simulink model "Bilanciamento_MPC"  (R2026b)
settings: Solver=FixedStepDiscrete  StartTime=0  StopTime=par_sim.t_fine  FixedStep=par_sim.Tint
PostLoadFcn:
  | addpath(genpath(fileparts(fileparts(get_param('Bilanciamento_MPC', 'FileName')))));
  | if ~evalin('base', 'exist(''par_sim'', ''var'')')
  |     assignin('base', 'par_sim', parametri_simulazione());
  | end
InitFcn:
  | addpath(genpath(fileparts(fileparts(get_param('Bilanciamento_MPC', 'FileName')))));
  | if ~evalin('base', 'exist(''par_sim'', ''var'')')
  |     assignin('base', 'par_sim', parametri_simulazione());
  | end
values from neighbouring files (symbols this model uses):
  par_sim = parametri_simulazione(par, pacco, formulazione, par.(['scenario' scenario]), orizzonte)    [avvio_simulink.m]    (also in simula_simulink.m = parametri_simulazione(par, pacco, tipo, scen, p))
libraries: simulink x2
settings Model: Creator=Acer  LastModifiedBy=Acer

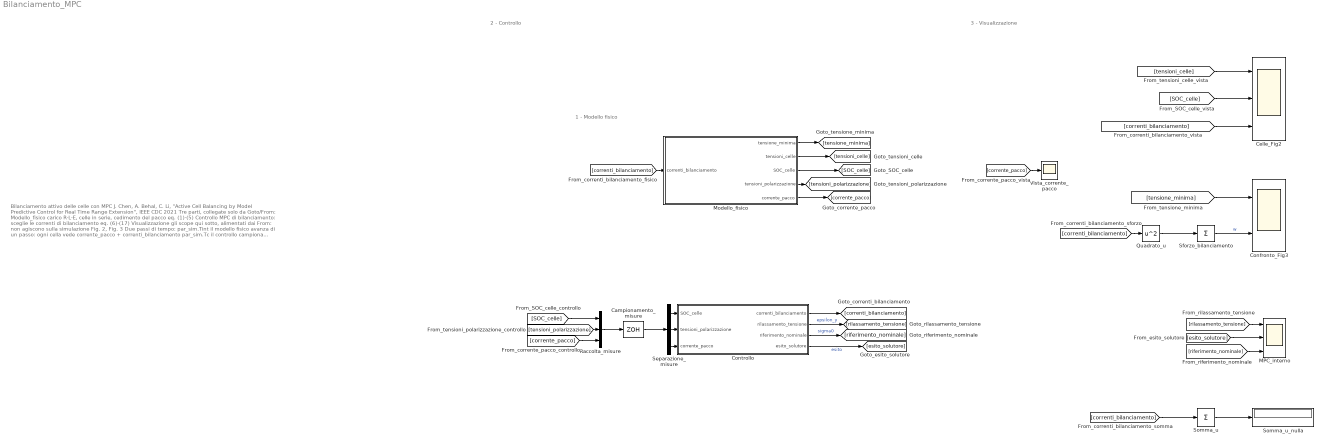
== system Bilanciamento_MPC ==
  note: Bilanciamento attivo delle celle con MPC
      | J. Chen, A. Behal, C. Li, "Active Cell Balancing by Model Predictive Control for Real Time Range Extension", IEEE CDC 2021
      |
      | Tre parti, collegate solo da Goto/From:
      |    Modello_fisico     carico R-L-E, celle in serie, cedimento del pacco             eq. (1)-(5)
      |    Controllo          MPC di bilanciamento: sceglie le correnti di bilanciamento    eq. (6)-(17)
      |    Visualizzazione    gli scope qui sotto, alimentati dai From: non agiscono sulla simulazione   Fig. 2, Fig. 3
      |
      | Due passi di tempo:
      |    par_sim.Tint         il modello fisico avanza di un passo: ogni cella vede corrente_pacco + correnti_bilanciamento
      |    par_sim.Tc           il controllo campiona corrente_pacco, SOC_celle e tensioni_polarizzazione e sceglie correnti_bilanciamento,
      |                         che restano costanti fino al passo di controllo successivo
      | La simulazione si ferma quando una cella scende sotto y_min.
      |
      | Parametri della simulazione nella struct 'par_sim' (avvio_simulink.m).
      | par_sim.n_J: 1 = J_t   2 = J_m   3 = J_Delta.  Confronto dei quattro casi: main_simulink.m
  note: 1 - Modello fisico
  note: 2 - Controllo
  note: 3 - Visualizzazione
  Campionamento_misure : ZeroOrderHold  SampleTime=par_sim.Tc
      settings: AttributesFormatString=ogni Tc
  Celle_Fig2 : Scope  NumInputPorts=3
      settings: AttributesFormatString=Fig. 2: y, s, u  ActiveDisplayString=3  Title=Corrente di bilanciamento u^n [A]  ActiveDisplayYMinimum=-2.4917702044223984  ActiveDisplayYMaximum=2.42593183980159
  Confronto_Fig3 : Scope  NumInputPorts=2
      settings: AttributesFormatString=Fig. 3: min y, sforzo w  Title=Sforzo di bilanciamento e_k = u_k'u_k [A^2]  ActiveDisplayYMinimum=0.52817346836693146  ActiveDisplayYMaximum=4.5629080222727767  DataLoggingVariableName=ScopeData2
  Controllo : Subsystem
      settings: AttributesFormatString=MPC: problema (6) risolto\ncome QP (Remark 3)
  MPC_interno : Scope  NumInputPorts=3
      settings: AttributesFormatString=epsilon_y, esito, sigma0  ActiveDisplayString=3  Title=Riferimento della cella nominale sigma0, eq. (7): una linea per passo dell'orizzonte  ActiveDisplayYMinimum=3.7199020855689335  ActiveDisplayYMaximum=4.2453442127145626
  Modello_fisico : Subsystem
      settings: AttributesFormatString=carico, celle, cedimento\neq. (1)-(5)
  Quadrato_u : Math  Operator=square
  Raccolta_misure : Mux  Inputs=[par_sim.N par_sim.N 1]
  Separazione_misure : Demux  Outputs=[par_sim.N par_sim.N 1]
  Sforzo_bilanciamento : Sum  Inputs=+
  Somma_u : Sum  Inputs=+
      settings: AttributesFormatString=eq. (6f)
  Somma_u_nulla : Display
      settings: AttributesFormatString=deve restare 0
  Vista_corrente_pacco : Scope
      settings: ActiveDisplayYMinimum=-2.0757062717769164  ActiveDisplayYMaximum=18.68135644599225  DataLoggingVariableName=ScopeData3
  wires:
  [correnti_bilanciamento] -> Quadrato_u/1
  Quadrato_u/1 -> Sforzo_bilanciamento/1
  [correnti_bilanciamento] -> Somma_u/1
  [correnti_bilanciamento] -> Celle_Fig2/3
  [riferimento_nominale] -> MPC_interno/3
  [esito_solutore] -> MPC_interno/2
  [SOC_celle] -> Celle_Fig2/2
  [rilassamento_tensione] -> MPC_interno/1
  [tensioni_celle] -> Celle_Fig2/1
  Sforzo_bilanciamento/1 -> Confronto_Fig3/2  "w"
  [tensione_minima] -> Confronto_Fig3/1
  Somma_u/1 -> Somma_u_nulla/1
  Controllo/4(esito_solutore) -> [esito_solutore]  "esito"
  Controllo/3(riferimento_nominale) -> [riferimento_nominale]  "sigma0"
  Controllo/2(rilassamento_tensione) -> [rilassamento_tensione]  "epsilon_y"
  Controllo/1(correnti_bilanciamento) -> [correnti_bilanciamento]
  Modello_fisico/5(corrente_pacco) -> [corrente_pacco]
  Modello_fisico/4(tensioni_polarizzazione) -> [tensioni_polarizzazione]
  Modello_fisico/3(SOC_celle) -> [SOC_celle]
  Modello_fisico/2(tensioni_celle) -> [tensioni_celle]
  Modello_fisico/1(tensione_minima) -> [tensione_minima]
  [correnti_bilanciamento] -> Modello_fisico/1(correnti_bilanciamento)
  [corrente_pacco] -> Vista_corrente_pacco/1
  [tensioni_polarizzazione] -> Raccolta_misure/2
  [SOC_celle] -> Raccolta_misure/1
  [corrente_pacco] -> Raccolta_misure/3
  Raccolta_misure/1 -> Campionamento_misure/1
  Campionamento_misure/1 -> Separazione_misure/1
  Separazione_misure/3 -> Controllo/3(corrente_pacco)
  Separazione_misure/2 -> Controllo/2(tensioni_polarizzazione)
  Separazione_misure/1 -> Controllo/1(SOC_celle)

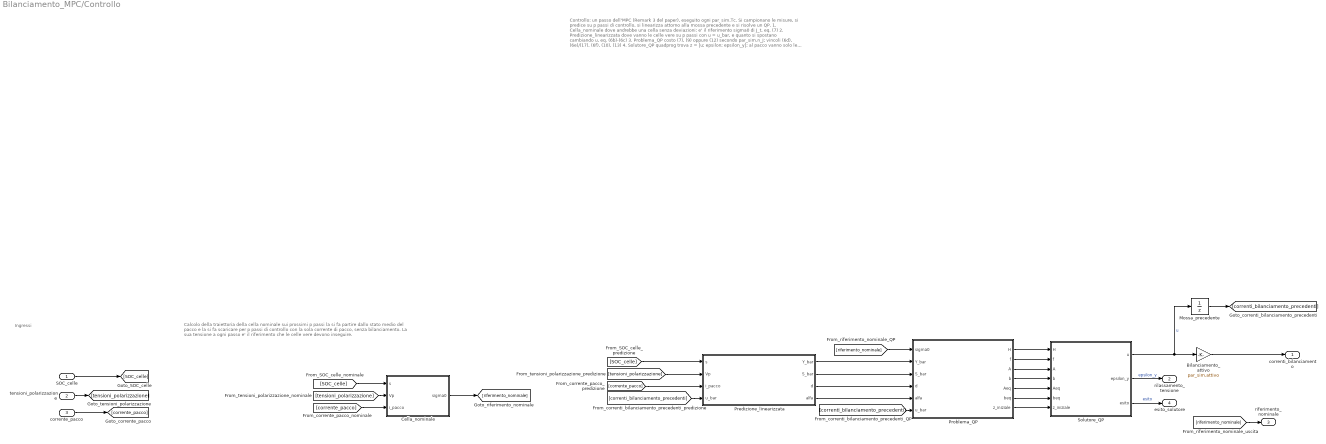
== system Bilanciamento_MPC/Controllo ==
  note: Ingressi
  note: Calcolo della traiettoria della cella nominale sui prossimi p passi
      |
      | la si fa partire dallo stato medio del pacco e la si fa scaricare per p passi di controllo con la sola corrente di pacco, senza bilanciamento.
      | La sua tensione a ogni passo e' il riferimento che le celle vere devono inseguire.
  note: Controllo: un passo dell'MPC (Remark 3 del paper), eseguito ogni par_sim.Tc. Si campionano le misure, si predice su p passi di controllo,
      | si linearizza attorno alla mossa precedente e si risolve un QP.
      |
      | 1. Cella_nominale            dove andrebbe una cella senza deviazioni: e' il riferimento sigma0 di J_t, eq. (7)
      | 2. Predizione_linearizzata   dove vanno le celle vere su p passi con u = u_bar, e quanto si spostano cambiando u, eq. (6b)-(6c)
      | 3. Problema_QP               costo (7), (9) oppure (12) secondo par_sim.n_J; vincoli (6d), (6e)/(17), (6f), (10), (13)
      | 4. Solutore_QP               quadprog trova z = [u; epsilon; epsilon_y]; al pacco vanno solo le u (orizzonte mobile)
      | 5. Bilanciamento_attivo      guadagno par_sim.attivo: con 0 il pacco lavora senza bilanciamento
      |
      | Doppio clic su un blocco per leggerne il codice; il calcolo vero e' nel file qp_*.m indicato nel commento.
  SOC_celle : Inport
  tensioni_polarizzazione : Inport  Port=2
  corrente_pacco : Inport  Port=3
  Bilanciamento_attivo : Gain  Gain=par_sim.attivo
      settings: AttributesFormatString=par_sim.attivo: 0 o 1
  Cella_nominale : MATLAB Function  TreatAsAtomicUnit=on
      settings: AttributesFormatString=eq. (7): riferimento sigma0
  Mossa_precedente : UnitDelay  InitialCondition=zeros(par_sim.N, 1)  SampleTime=par_sim.Tc
      settings: AttributesFormatString=u_bar = u_(k-1)
  Predizione_linearizzata : MATLAB Function  TreatAsAtomicUnit=on
      settings: AttributesFormatString=eq. (6b)-(6c), Remark 3
  Problema_QP : MATLAB Function  TreatAsAtomicUnit=on
      settings: AttributesFormatString=costo (7)/(9)/(12) e vincoli
  Solutore_QP : MATLAB Function  TreatAsAtomicUnit=on
      settings: AttributesFormatString=quadprog
  correnti_bilanciamento : Outport
  rilassamento_tensione : Outport  Port=2
  riferimento_nominale : Outport  Port=3
  esito_solutore : Outport  Port=4
  wires:
  corrente_pacco/1 -> [corrente_pacco]
  [corrente_pacco] -> Predizione_linearizzata/3(i_pacco)
  [tensioni_polarizzazione] -> Predizione_linearizzata/2(Vp)
  [SOC_celle] -> Predizione_linearizzata/1(s)
  [corrente_pacco] -> Cella_nominale/3(i_pacco)
  [tensioni_polarizzazione] -> Cella_nominale/2(Vp)
  [SOC_celle] -> Cella_nominale/1(s)
  Cella_nominale/1(sigma0) -> [riferimento_nominale]
  Predizione_linearizzata/1(Y_bar) -> Problema_QP/2(Y_bar)
  Predizione_linearizzata/2(S_bar) -> Problema_QP/3(S_bar)
  Predizione_linearizzata/3(d) -> Problema_QP/4(d)
  Predizione_linearizzata/4(alfa) -> Problema_QP/5(alfa)
  Problema_QP/1(H) -> Solutore_QP/1(H)
  Problema_QP/2(f) -> Solutore_QP/2(f)
  Problema_QP/3(A) -> Solutore_QP/3(A)
  Problema_QP/4(b) -> Solutore_QP/4(b)
  Problema_QP/5(Aeq) -> Solutore_QP/5(Aeq)
  Problema_QP/6(beq) -> Solutore_QP/6(beq)
  Problema_QP/7(z_iniziale) -> Solutore_QP/7(z_iniziale)
  [correnti_bilanciamento_precedenti] -> Predizione_linearizzata/4(u_bar)
  [correnti_bilanciamento_precedenti] -> Problema_QP/6(u_bar)
  Mossa_precedente/1 -> [correnti_bilanciamento_precedenti]
  Bilanciamento_attivo/1 -> correnti_bilanciamento/1
  Solutore_QP/1(u) -> Mossa_precedente/1, Bilanciamento_attivo/1  "u"
  tensioni_polarizzazione/1 -> [tensioni_polarizzazione]
  SOC_celle/1 -> [SOC_celle]
  [riferimento_nominale] -> riferimento_nominale/1
  [riferimento_nominale] -> Problema_QP/1(sigma0)
  Solutore_QP/2(epsilon_y) -> rilassamento_tensione/1  "epsilon_y"
  Solutore_QP/3(esito) -> esito_solutore/1  "esito"

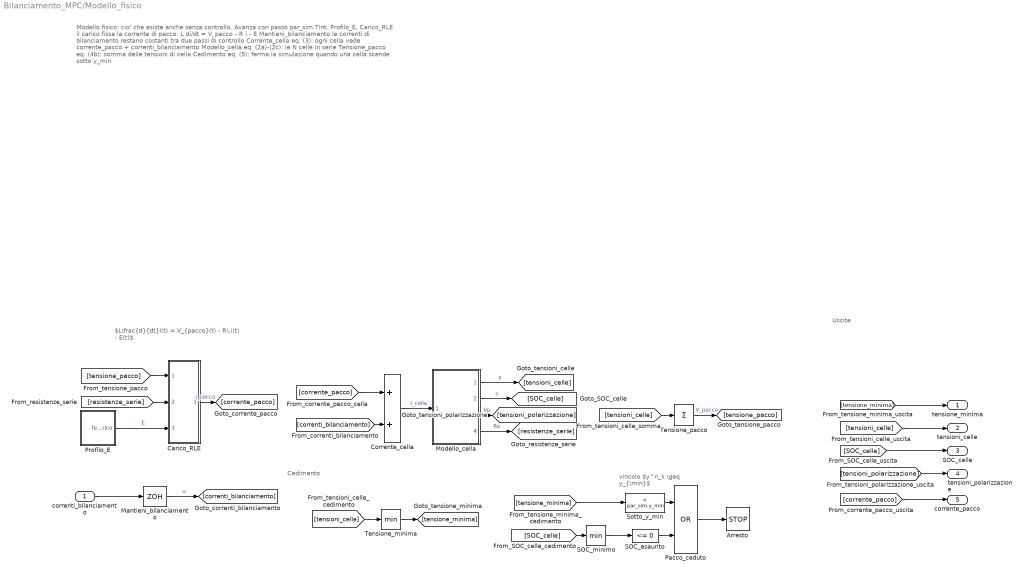
== system Bilanciamento_MPC/Modello_fisico ==
  note: vincolo $y^n_k \geq y_{\min}$
  note: $L\frac{d}{dt}i(t) = V_{pacco}(t) - R\,i(t) - E(t)$
  note: Cedimento
  note: Uscite
  note: Modello fisico: cio' che esiste anche senza controllo. Avanza con passo par_sim.Tint.
      |
      |    Profilo_E, Carico_RLE   il carico fissa la corrente di pacco:  L di/dt = V_pacco - R i - E
      |    Mantieni_bilanciamento  le correnti di bilanciamento restano costanti tra due passi di controllo
      |    Corrente_cella          eq. (3): ogni cella vede corrente_pacco + correnti_bilanciamento
      |    Modello_cella           eq. (2a)-(2c): le N celle in serie
      |    Tensione_pacco          eq. (4b): somma delle tensioni di cella
      |    Cedimento               eq. (5): ferma la simulazione quando una cella scende sotto y_min
  correnti_bilanciamento : Inport
  Arresto : Stop
  Carico_RLE : Subsystem
      settings: AttributesFormatString=L di_pacco/dt = V_pacco - R i_pacco - E
  Corrente_cella : Sum
      settings: AttributesFormatString=eq. (3): I_cella = i_pacco + u
  Mantieni_bilanciamento : ZeroOrderHold  SampleTime=par_sim.Tint
      settings: AttributesFormatString=costante tra due passi\ndi controllo
  Modello_cella : Subsystem
      settings: AttributesFormatString=eq. (2a)-(2c), (4a)
  Pacco_ceduto : Logic  Operator=OR  AllPortsSameDT=off  OutDataTypeStr=boolean
  Profilo_E : Subsystem
      settings: AttributesFormatString=f.e.m. del carico E(t)
  SOC_esaurito : simulink/Logic and Bit Operations/Compare To Constant  relop=<=  const=0  OutDataTypeStr=boolean
  SOC_minimo : MinMax
  Sotto_y_min : simulink/Logic and Bit Operations/Compare To Constant  relop=<  const=par_sim.y_min  OutDataTypeStr=boolean
  Tensione_minima : MinMax
  Tensione_pacco : Sum  Inputs=+
      settings: AttributesFormatString=eq. (4b)
  tensione_minima : Outport
  tensioni_celle : Outport  Port=2
  SOC_celle : Outport  Port=3
  tensioni_polarizzazione : Outport  Port=4
  corrente_pacco : Outport  Port=5
  wires:
  correnti_bilanciamento/1 -> Mantieni_bilanciamento/1
  [tensioni_celle] -> Tensione_pacco/1
  Modello_cella/1(tensioni_celle) -> [tensioni_celle]  "y"
  [correnti_bilanciamento] -> Corrente_cella/2
  [tensione_pacco] -> Carico_RLE/1(tensione_pacco)
  Modello_cella/2(SOC_celle) -> [SOC_celle]  "s"
  Tensione_pacco/1 -> [tensione_pacco]  "V_pacco"
  [resistenze_serie] -> Carico_RLE/2(resistenze_serie)
  Modello_cella/4(resistenze_serie) -> [resistenze_serie]  "Ro"
  Profilo_E/1(fem_carico) -> Carico_RLE/3(fem_carico)  "E"
  Corrente_cella/1 -> Modello_cella/1(correnti_celle)  "I_cella"
  Carico_RLE/1(corrente_pacco) -> [corrente_pacco]  "i_pacco"
  [corrente_pacco] -> Corrente_cella/1
  Mantieni_bilanciamento/1 -> [correnti_bilanciamento]  "u"
  [corrente_pacco] -> corrente_pacco/1
  [tensione_minima] -> tensione_minima/1
  [SOC_celle] -> SOC_celle/1
  Modello_cella/3(tensioni_polarizzazione) -> [tensioni_polarizzazione]  "Vp"
  [tensioni_polarizzazione] -> tensioni_polarizzazione/1
  [tensioni_celle] -> tensioni_celle/1
  Sotto_y_min/1 -> Pacco_ceduto/1
  [tensione_minima] -> Sotto_y_min/1
  SOC_minimo/1 -> SOC_esaurito/1
  Pacco_ceduto/1 -> Arresto/1
  [SOC_celle] -> SOC_minimo/1
  SOC_esaurito/1 -> Pacco_ceduto/2
  [tensioni_celle] -> Tensione_minima/1
  Tensione_minima/1 -> [tensione_minima]

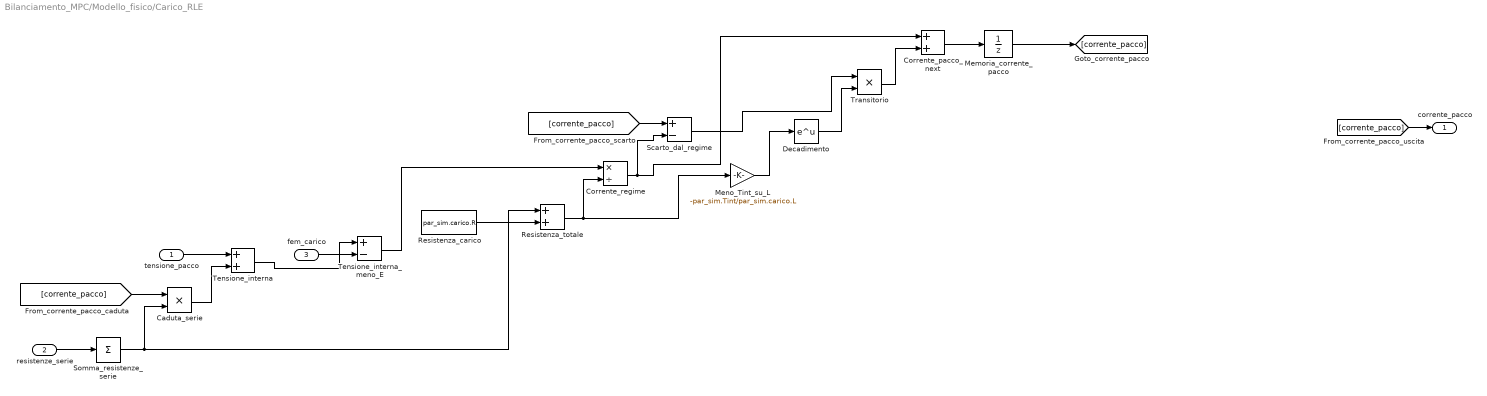
== system Bilanciamento_MPC/Modello_fisico/Carico_RLE ==
  tensione_pacco : Inport
  resistenze_serie : Inport  Port=2
  fem_carico : Inport  Port=3
  Caduta_serie : Product  Inputs=**
  Corrente_pacco_next : Sum
  Corrente_regime : Product  Inputs=*/
      settings: AttributesFormatString=(V_int - E) / R_tot
  Decadimento : Math
      settings: AttributesFormatString=exp(-Tint*R_tot/L)
  Memoria_corrente_pacco : UnitDelay  InitialCondition=par_sim.i_pacco_iniziale  SampleTime=par_sim.Tint
      settings: AttributesFormatString=stato i_pacco
  Meno_Tint_su_L : Gain  Gain=-par_sim.Tint/par_sim.carico.L
  Resistenza_carico : Constant  Value=par_sim.carico.R  SampleTime=par_sim.Tint
  Resistenza_totale : Sum
  Scarto_dal_regime : Sum  Inputs=+-
  Somma_resistenze_serie : Sum  Inputs=+
  Tensione_interna : Sum
      settings: AttributesFormatString=tensione del pacco a i_pacco = 0
  Tensione_interna_meno_E : Sum  Inputs=+-
  Transitorio : Product  Inputs=**
  corrente_pacco : Outport
  wires:
  [corrente_pacco] -> Scarto_dal_regime/1
  [corrente_pacco] -> Caduta_serie/1
  resistenze_serie/1 -> Somma_resistenze_serie/1
  Somma_resistenze_serie/1 -> Caduta_serie/2, Resistenza_totale/1
  Resistenza_carico/1 -> Resistenza_totale/2
  Memoria_corrente_pacco/1 -> [corrente_pacco]
  tensione_pacco/1 -> Tensione_interna/1
  Caduta_serie/1 -> Tensione_interna/2
  Tensione_interna/1 -> Tensione_interna_meno_E/1
  fem_carico/1 -> Tensione_interna_meno_E/2
  Tensione_interna_meno_E/1 -> Corrente_regime/1
  Resistenza_totale/1 -> Meno_Tint_su_L/1, Corrente_regime/2
  Meno_Tint_su_L/1 -> Decadimento/1
  Corrente_regime/1 -> Corrente_pacco_next/1, Scarto_dal_regime/2
  Scarto_dal_regime/1 -> Transitorio/1
  Decadimento/1 -> Transitorio/2
  Transitorio/1 -> Corrente_pacco_next/2
  Corrente_pacco_next/1 -> Memoria_corrente_pacco/1
  [corrente_pacco] -> corrente_pacco/1

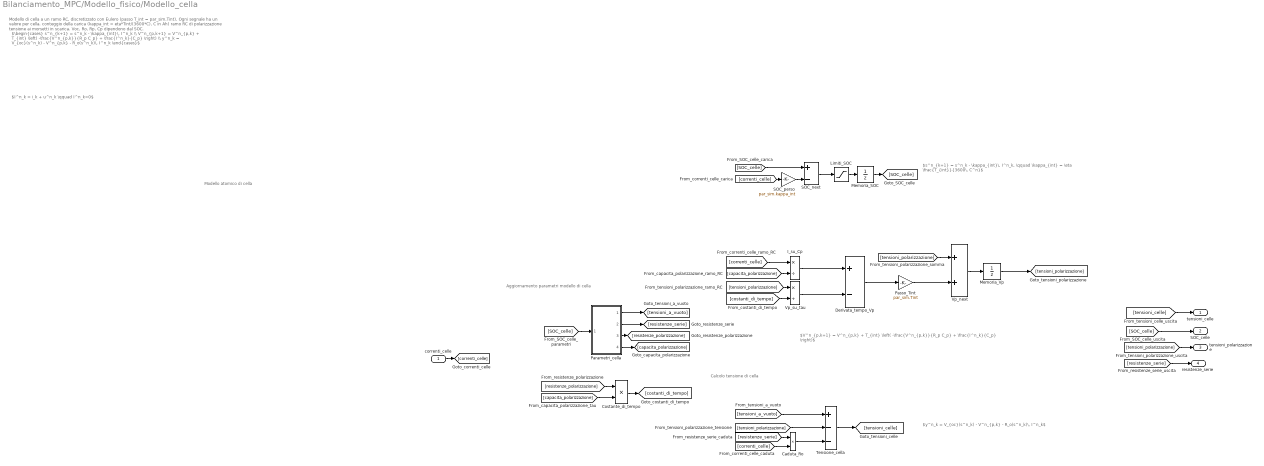
== system Bilanciamento_MPC/Modello_fisico/Modello_cella ==
  note: Modello atomico di cella
  note: $I^n_k = i_k + u^n_k \qquad I^n_k>0$
  note: $\begin{cases} s^n_{k+1} = s^n_k - \kappa_{int}\, I^n_k \\ V^n_{p,k+1} = V^n_{p,k} + T_{int} \left( -\frac{V^n_{p,k}}{R_p C_p} + \frac{I^n_k}{C_p} \right) \\ y^n_k = V_{oc}(s^n_k) - V^n_{p,k} - R_o(s^n_k)\, I^n_k \end{cases}$
  note: Calcolo tensione di cella
  note: Aggiornamento parametri modello di cella
  note: Modello di cella a un ramo RC, discretizzato con Eulero (passo T_int = par_sim.Tint). Ogni segnale ha un valore per cella.
      |
      | conteggio della carica (kappa_int = eta*Tint/(3600*C), C in Ah)
      |
      | ramo RC di polarizzazione
      |
      | tensione ai morsetti
      |
      | in scarica. Voc, Ro, Rp, Cp dipendono dal SOC.
  note: $V^n_{p,k+1} = V^n_{p,k} + T_{int} \left( -\frac{V^n_{p,k}}{R_p C_p} + \frac{I^n_k}{C_p} \right)$
  note: $y^n_k = V_{oc}(s^n_k) - V^n_{p,k} - R_o(s^n_k)\, I^n_k$
  note: $s^n_{k+1} = s^n_k - \kappa_{int}\, I^n_k, \qquad \kappa_{int} = \eta \frac{T_{int}}{3600\, C^n}$
  correnti_celle : Inport
  Caduta_Ro : Product  Inputs=**
  Costante_di_tempo : Product  Inputs=**
  Derivata_tempo_Vp : Sum  Inputs=+-
  I_su_Cp : Product  Inputs=*/
  Limiti_SOC : Saturate  UpperLimit=1  LowerLimit=0
  Memoria_SOC : UnitDelay  InitialCondition=par_sim.s_iniziale  SampleTime=par_sim.Tint
      settings: AttributesFormatString=stato s
  Memoria_Vp : UnitDelay  InitialCondition=par_sim.Vp_iniziale  SampleTime=par_sim.Tint
      settings: AttributesFormatString=stato V_p
  Parametri_cella : Subsystem
      settings: AttributesFormatString=V_oc, R_o, R_p, C_p(SOC)
  Passo_Tint : Gain  Gain=par_sim.Tint
  SOC_next : Sum  Inputs=+-
  SOC_perso : Gain  Gain=par_sim.kappa_int
      settings: AttributesFormatString=kappa_int * I_cella
  Tensione_cella : Sum  Inputs=+--
      settings: AttributesFormatString=eq. (2c)
  Vp_next : Sum
      settings: AttributesFormatString=eq. (2b)
  Vp_su_tau : Product  Inputs=*/
  tensioni_celle : Outport
  SOC_celle : Outport  Port=2
  tensioni_polarizzazione : Outport  Port=3
  resistenze_serie : Outport  Port=4
  wires:
  correnti_celle/1 -> [correnti_celle]
  [tensioni_polarizzazione] -> Vp_next/1
  [tensioni_polarizzazione] -> Vp_su_tau/1
  [tensioni_polarizzazione] -> Tensione_cella/2
  [SOC_celle] -> SOC_celle/1
  [SOC_celle] -> SOC_next/1
  [correnti_celle] -> I_su_Cp/1
  [correnti_celle] -> SOC_perso/1
  [correnti_celle] -> Caduta_Ro/2
  Vp_next/1 -> Memoria_Vp/1
  Passo_Tint/1 -> Vp_next/2
  Derivata_tempo_Vp/1 -> Passo_Tint/1
  Vp_su_tau/1 -> Derivata_tempo_Vp/2
  I_su_Cp/1 -> Derivata_tempo_Vp/1
  Limiti_SOC/1 -> Memoria_SOC/1
  SOC_next/1 -> Limiti_SOC/1
  SOC_perso/1 -> SOC_next/2
  Caduta_Ro/1 -> Tensione_cella/3
  Memoria_Vp/1 -> [tensioni_polarizzazione]
  Memoria_SOC/1 -> [SOC_celle]
  [SOC_celle] -> Parametri_cella/1(SOC_celle)
  [resistenze_serie] -> resistenze_serie/1
  [resistenze_serie] -> Caduta_Ro/1
  Parametri_cella/2(resistenze_serie) -> [resistenze_serie]
  [resistenze_polarizzazione] -> Costante_di_tempo/1
  Parametri_cella/3(resistenze_polarizzazione) -> [resistenze_polarizzazione]
  Parametri_cella/4(capacita_polarizzazione) -> [capacita_polarizzazione]
  [capacita_polarizzazione] -> Costante_di_tempo/2
  [capacita_polarizzazione] -> I_su_Cp/2
  [tensioni_a_vuoto] -> Tensione_cella/1
  Parametri_cella/1(tensioni_a_vuoto) -> [tensioni_a_vuoto]
  Costante_di_tempo/1 -> [costanti_di_tempo]
  [costanti_di_tempo] -> Vp_su_tau/2
  [tensioni_polarizzazione] -> tensioni_polarizzazione/1
  [tensioni_celle] -> tensioni_celle/1
  Tensione_cella/1 -> [tensioni_celle]

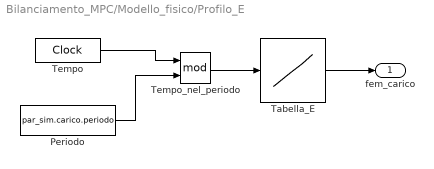
== system Bilanciamento_MPC/Modello_fisico/Profilo_E ==
  Periodo : Constant  Value=par_sim.carico.periodo  SampleTime=par_sim.Tint
  Tabella_E : Lookup_n-D  NumberOfTableDimensions=1  BreakpointsForDimension1=par_sim.carico.t_E  Table=par_sim.carico.E  ExtrapMethod=Clip  InternalRulePriority=Speed  RndMeth=Simplest
  Tempo : DigitalClock  SampleTime=par_sim.Tint
  Tempo_nel_periodo : Math  Operator=mod
  fem_carico : Outport
  wires:
  Tempo/1 -> Tempo_nel_periodo/1
  Periodo/1 -> Tempo_nel_periodo/2
  Tempo_nel_periodo/1 -> Tabella_E/1
  Tabella_E/1 -> fem_carico/1

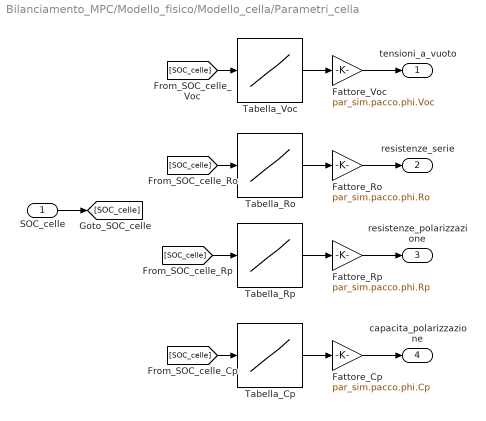
== system Bilanciamento_MPC/Modello_fisico/Modello_cella/Parametri_cella ==
  SOC_celle : Inport
  Fattore_Cp : Gain  Gain=par_sim.pacco.phi.Cp
  Fattore_Ro : Gain  Gain=par_sim.pacco.phi.Ro
  Fattore_Rp : Gain  Gain=par_sim.pacco.phi.Rp
  Fattore_Voc : Gain  Gain=par_sim.pacco.phi.Voc
  Tabella_Cp : Lookup_n-D  NumberOfTableDimensions=1  BreakpointsForDimension1=par_sim.pacco.s_tab  Table=par_sim.pacco.Cp_tab  ExtrapMethod=Clip  InternalRulePriority=Speed  RndMeth=Simplest
  Tabella_Ro : Lookup_n-D  NumberOfTableDimensions=1  BreakpointsForDimension1=par_sim.pacco.s_tab  Table=par_sim.pacco.Ro_tab  ExtrapMethod=Clip  InternalRulePriority=Speed  RndMeth=Simplest
  Tabella_Rp : Lookup_n-D  NumberOfTableDimensions=1  BreakpointsForDimension1=par_sim.pacco.s_tab  Table=par_sim.pacco.Rp_tab  ExtrapMethod=Clip  InternalRulePriority=Speed  RndMeth=Simplest
  Tabella_Voc : Lookup_n-D  NumberOfTableDimensions=1  BreakpointsForDimension1=par_sim.pacco.s_tab  Table=par_sim.pacco.Voc_tab  ExtrapMethod=Clip  InternalRulePriority=Speed  RndMeth=Simplest
  tensioni_a_vuoto : Outport
  resistenze_serie : Outport  Port=2
  resistenze_polarizzazione : Outport  Port=3
  capacita_polarizzazione : Outport  Port=4
  wires:
  Tabella_Voc/1 -> Fattore_Voc/1
  Tabella_Ro/1 -> Fattore_Ro/1
  Tabella_Rp/1 -> Fattore_Rp/1
  Tabella_Cp/1 -> Fattore_Cp/1
  Fattore_Voc/1 -> tensioni_a_vuoto/1
  Fattore_Ro/1 -> resistenze_serie/1
  Fattore_Rp/1 -> resistenze_polarizzazione/1
  Fattore_Cp/1 -> capacita_polarizzazione/1
  SOC_celle/1 -> [SOC_celle]
  [SOC_celle] -> Tabella_Rp/1
  [SOC_celle] -> Tabella_Cp/1
  [SOC_celle] -> Tabella_Voc/1
  [SOC_celle] -> Tabella_Ro/1

== matlab function Bilanciamento_MPC/Controllo/Predizione_linearizzata ==
  data: s input; Y_bar output; Vp input; i_pacco input; u_bar input; S_bar output; d output; alfa output; par_sim parameter
function [Y_bar, S_bar, d, alfa] = Predizione_linearizzata(s, Vp, i_pacco, u_bar, par_sim)
% Modello di predizione, eq. (6b)-(6c), linearizzato come nel Remark 3.
%
% Integra le celle per p passi di controllo con la corrente i_pacco + u_bar tenuta
% costante (u_bar e' la mossa precedente) e calcola i coefficienti di sensibilita'
% rispetto a u:
%   y_{k+j}(u) ~= Y_bar(j,:) + d(j,:)    .* (u - u_bar)
%   s_{k+j}(u) ~= S_bar(j,:) + alfa(j,:) .* (u - u_bar)
% Y_bar, S_bar, d, alfa sono p x N: riga j <-> istante k+j, colonna n <-> cella n.
%
% Codice: qp_predizione.m

[Y_bar, S_bar, d, alfa] = qp_predizione(par_sim.pacco, s, Vp, i_pacco + u_bar, par_sim.p, par_sim.Tc);

== matlab function Bilanciamento_MPC/Controllo/Cella_nominale ==
  data: s input; sigma0 output; Vp input; i_pacco input; par_sim parameter
function sigma0 = Cella_nominale(s, Vp, i_pacco, par_sim)
% Riferimento per J_t, eq. (7) del paper.
%
% La cella nominale (parametri senza deviazione) parte dalla media degli stati
% del pacco e viene integrata su p passi con la sola corrente di pacco i_pacco.
% sigma0 e' p x 1: riga j <-> istante k+j.
%
% Codice: cella_nominale_semplice.m

sigma0 = cella_nominale_semplice(par_sim, s, Vp, i_pacco);

== matlab function Bilanciamento_MPC/Controllo/Problema_QP ==
  data: sigma0 input; H output; Y_bar input; S_bar input; d input; alfa input; u_bar input; f output; A output; b output; Aeq output; beq output; z_iniziale output; par_sim parameter
function [H, f, A, b, Aeq, beq, z_iniziale] = Problema_QP(sigma0, Y_bar, S_bar, d, alfa, u_bar, par_sim)
% Il problema (6) del paper scritto come QP nelle incognite z = [u; epsilon; epsilon_y]:
%
%   min 1/2*z'*H*z + f'*z    con  A*z <= b,  Aeq*z = beq
%
%   H, f        costo: (7) per Jt, (9) per Jm, (12) per Jdelta, piu' rho*u'*u e W*epsilon_y^2
%   A, b        (6e) rilassata come in (17), (10)/(13) sulle epsilon, limiti (6d)
%   Aeq, beq    (6f): somma delle u nulla
%   z_iniziale  punto di partenza: la mossa del passo precedente
%
% Codice: qp_problema.m

[H, f, A, b, Aeq, beq, z_iniziale] = qp_problema(par_sim, sigma0, Y_bar, S_bar, d, alfa, u_bar);

== matlab function Bilanciamento_MPC/Controllo/Solutore_QP ==
  data: H input; u output; epsilon_y output; f input; A input; b input; Aeq input; beq input; z_iniziale input; esito output; par_sim parameter
function [u, epsilon_y, esito] = Solutore_QP(H, f, A, b, Aeq, beq, z_iniziale, par_sim)
% Risolve il QP con quadprog, come nel paper (Sez. IV-A), e applica solo le
% correnti di bilanciamento u (orizzonte mobile).
%
%   min  1/2*z'*H*z + f'*z     con  A*z <= b,  Aeq*z = beq
%
%   u          prime N componenti di z: le correnti da applicare al passo k
%   epsilon_y  ultima componente di z: variabile di rilassamento del vincolo di tensione, eq. (17)
%   esito      exitflag di quadprog (1 = soluzione trovata)
%
% z_iniziale e' il punto di partenza ammissibile costruito da qp_problema con la
% mossa del passo precedente: se quadprog non trova una soluzione,
% z = z_iniziale e la mossa precedente viene mantenuta.
%
% Codice: qp_solutore.m

persistent opzioni
if isempty(opzioni)
    % 'active-set' si ferma su un vertice esatto: adatto a Jm e Jdelta, che
    % nelle variabili ausiliarie epsilon sono problemi lineari
    opzioni = optimoptions('quadprog', 'Algorithm', 'active-set', 'Display', 'off');
end

[z, ~, esito] = quadprog(H, f, A, b, Aeq, beq, [], [], z_iniziale, opzioni);

if esito <= 0 || isempty(z)
    z = z_iniziale;
end

u = z(1:par_sim.N);
epsilon_y = z(end);
